simulink model "SC_Stage_Detail"  (R2026a)
settings: Solver=daessc  StopTime=Pd.Tend  MaxStep=1/(50*Pd.f)  RelTol=1e-5
undefined symbols (not defined in the file): Pd
libraries: fl_lib x8, nesl_utility x7, ee_lib x4
settings Model: Creator=highdreameater  LastModifiedBy=highdreameater

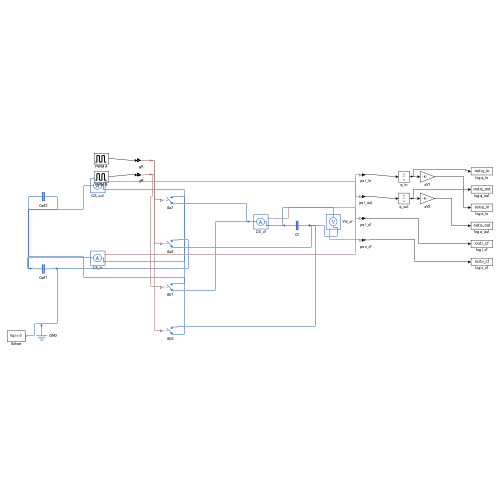
[thumbnail: Simulink's stored preview of the top-level diagram]
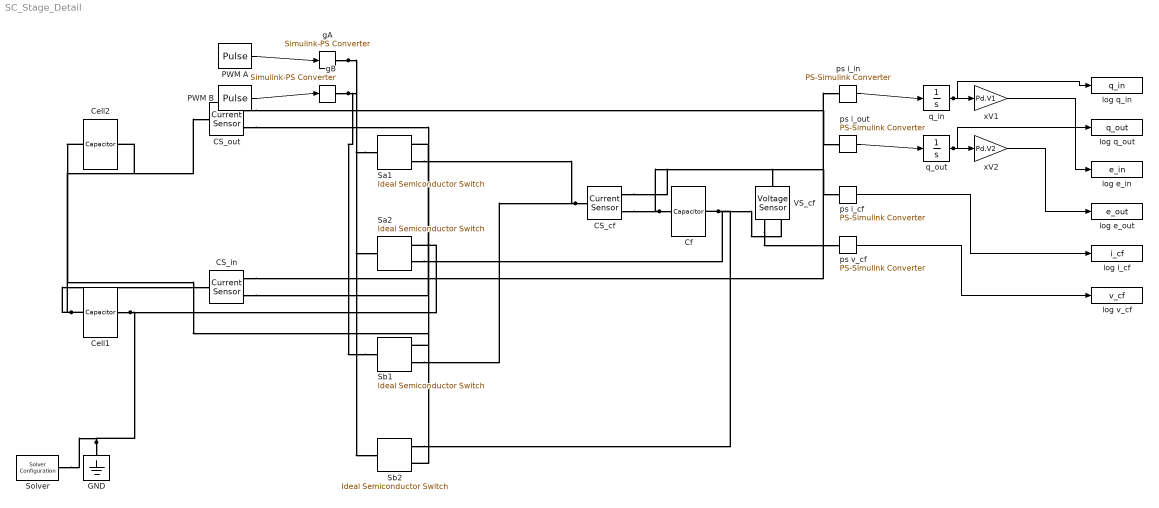
== system SC_Stage_Detail ==
  CS_cf : fl_lib/Electrical/Electrical Sensors/Current Sensor
  CS_in : fl_lib/Electrical/Electrical Sensors/Current Sensor
  CS_out : fl_lib/Electrical/Electrical Sensors/Current Sensor
  Cell1 : fl_lib/Electrical/Electrical Elements/Capacitor  c=Pd.C_emu F  r=Pd.ESR_emu Ohm  g=0 1/Ohm  i_specify=off  i_priority=None  i=0 A  i_nominal_specify=off  i_nominal_value=1  i_nominal_unit=A  v_specify=off  v_priority=None  v=0 V  v_nominal_specify=off  v_nominal_value=1  v_nominal_unit=V  vc_specify=on  vc_priority=High  vc=Pd.V1 V  vc_nominal_specify=off  vc_nominal_value=1  vc_nominal_unit=V
  Cell2 : fl_lib/Electrical/Electrical Elements/Capacitor  c=Pd.C_emu F  r=Pd.ESR_emu Ohm  g=0 1/Ohm  i_specify=off  i_priority=None  i=0 A  i_nominal_specify=off  i_nominal_value=1  i_nominal_unit=A  v_specify=off  v_priority=None  v=0 V  v_nominal_specify=off  v_nominal_value=1  v_nominal_unit=V  vc_specify=on  vc_priority=High  vc=Pd.V2 V  vc_nominal_specify=off  vc_nominal_value=1  vc_nominal_unit=V
  Cf : fl_lib/Electrical/Electrical Elements/Capacitor  c=Pd.C_fly F  r=Pd.ESR_fly Ohm  g=0 1/Ohm  i_specify=off  i_priority=None  i=0 A  i_nominal_specify=off  i_nominal_value=1  i_nominal_unit=A  v_specify=off  v_priority=None  v=0 V  v_nominal_specify=off  v_nominal_value=1  v_nominal_unit=V  vc_specify=on  vc_priority=High  vc=(Pd.V1+Pd.V2)/2 V  vc_nominal_specify=off  vc_nominal_value=1  vc_nominal_unit=V
  GND : fl_lib/Electrical/Electrical Elements/Electrical Reference
  PWM A : DiscretePulseGenerator  PulseType=Time based  Period=1/Pd.f  PulseWidth=Pd.duty_sc*100
  PWM B : DiscretePulseGenerator  PulseType=Time based  Period=1/Pd.f  PulseWidth=Pd.duty_sc*100  PhaseDelay=0.5/Pd.f
  Sa1 : ee_lib/Semiconductors & Converters/Ideal Semiconductor Switch  port_option=ee.enum.controlport.ps  Ron=Pd.R_on_sc Ohm  Goff=1e-9 1/Ohm  Vth=0.5 V  diode_param=ee.enum.semiconductors.protectionDiode.external  diode_Vf=0.8 V  diode_Ron=0.001 Ohm  diode_Goff=1e-5 1/Ohm  diode_C=50e-9 F  diode_iRM=-235 A  diode_iF=300 A  diode_idot=-50 A/us  diode_trr_param=ee.enum.converters.diodetrr.trr_factor  diode_trr_factor=3  diode_trr=15 us  diode_Qrr=1500 s*uA
  Sa2 : ee_lib/Semiconductors & Converters/Ideal Semiconductor Switch  port_option=ee.enum.controlport.ps  Ron=Pd.R_on_sc Ohm  Goff=1e-9 1/Ohm  Vth=0.5 V  diode_param=ee.enum.semiconductors.protectionDiode.external  diode_Vf=0.8 V  diode_Ron=0.001 Ohm  diode_Goff=1e-5 1/Ohm  diode_C=50e-9 F  diode_iRM=-235 A  diode_iF=300 A  diode_idot=-50 A/us  diode_trr_param=ee.enum.converters.diodetrr.trr_factor  diode_trr_factor=3  diode_trr=15 us  diode_Qrr=1500 s*uA
  Sb1 : ee_lib/Semiconductors & Converters/Ideal Semiconductor Switch  port_option=ee.enum.controlport.ps  Ron=Pd.R_on_sc Ohm  Goff=1e-9 1/Ohm  Vth=0.5 V  diode_param=ee.enum.semiconductors.protectionDiode.external  diode_Vf=0.8 V  diode_Ron=0.001 Ohm  diode_Goff=1e-5 1/Ohm  diode_C=50e-9 F  diode_iRM=-235 A  diode_iF=300 A  diode_idot=-50 A/us  diode_trr_param=ee.enum.converters.diodetrr.trr_factor  diode_trr_factor=3  diode_trr=15 us  diode_Qrr=1500 s*uA
  Sb2 : ee_lib/Semiconductors & Converters/Ideal Semiconductor Switch  port_option=ee.enum.controlport.ps  Ron=Pd.R_on_sc Ohm  Goff=1e-9 1/Ohm  Vth=0.5 V  diode_param=ee.enum.semiconductors.protectionDiode.external  diode_Vf=0.8 V  diode_Ron=0.001 Ohm  diode_Goff=1e-5 1/Ohm  diode_C=50e-9 F  diode_iRM=-235 A  diode_iF=300 A  diode_idot=-50 A/us  diode_trr_param=ee.enum.converters.diodetrr.trr_factor  diode_trr_factor=3  diode_trr=15 us  diode_Qrr=1500 s*uA
  Solver : nesl_utility/Solver Configuration  PhysicalDomain=network_engine_domain  SubClassName=solver  LeftPortType=input  RightPortType=generic  Tones=[]  Harmonics=[]  SimulateNoise=off  Profile=off  UseLocalSampling=off  EnableSwitchedLinearOptims=on  FrequencyDomain=off  UseCCode=off  RelTol=0.001  AbsTol=0.001  MinStep=1e-09  ToWorkspace=off  RevertToSquareIcSolve=off  NumHomotopyIterations=100  PhasorMode=off  PhasorModeNumHarmonics=1  ConsistencySolver=NEWTON_XTOL_AFTER_FTOL  CanonicalOrdering=CANONICAL  OptimizeIntermediates=OPTIMIZED  IndexReductionMethod=DerivativeReplacement  DoDC=off  ResidualTolerance=1e-09  ConsistencyTolSource=GLOBAL  ConsistencyAbsTol=0.001  ConsistencyRelTol=0.001  ConsistencyTolFactor=0.001  UseLocalSolver=off  LocalSolverChoice=NE_BACKWARD_EULER_ADVANCER  ResolveIndetEquations=on  FunctionEvalNumThread=1  LocalSolverSampleTime=0.001  DoFixedCost=off  MaxNonlinIter=3  MaxModeIter=2  ComputeImpulses=off  ImpulseIterations=2  LinearAlgebra=auto  LinearAlgebraNumThread=0  EquationFormulation=NE_TIME_EF  DelaysMemoryBudget=1024  AutomaticFiltering=on  FilteringTimeConstant=0.001  PartitionStorageMethod=AS_NEEDED  PartitionMemoryBudget=1024  PartitionMethod=ROBUST  MultibodyUseLocalSolver=off  MultibodyLocalSolverChoice=ODE1  MultibodyLocalSolverSampleTime=0.001
  VS_cf : fl_lib/Electrical/Electrical Sensors/Voltage Sensor
  gA : nesl_utility/Simulink-PS Converter  PhysicalDomain=network_engine_domain  SubClassName=ps_input  LeftPortType=input  RightPortType=output  PseudoPeriodic=off  Frequencies=[]  NoiseDistribution=none  NoiseParameters=[]  Unit=1  AffineConversion=off  FilteringAndDerivatives=provide  SimscapeFilterOrder=1  InputFilterTimeConstant=0.001  UdotUserProvided=0
  gB : nesl_utility/Simulink-PS Converter  PhysicalDomain=network_engine_domain  SubClassName=ps_input  LeftPortType=input  RightPortType=output  PseudoPeriodic=off  Frequencies=[]  NoiseDistribution=none  NoiseParameters=[]  Unit=1  AffineConversion=off  FilteringAndDerivatives=provide  SimscapeFilterOrder=1  InputFilterTimeConstant=0.001  UdotUserProvided=0
  log e_in : ToWorkspace  VariableName=e_in  SaveFormat=Timeseries  SampleTime=-1
  log e_out : ToWorkspace  VariableName=e_out  SaveFormat=Timeseries  SampleTime=-1
  log i_cf : ToWorkspace  VariableName=i_cf  SaveFormat=Timeseries  SampleTime=-1
  log q_in : ToWorkspace  VariableName=q_in  SaveFormat=Timeseries  SampleTime=-1
  log q_out : ToWorkspace  VariableName=q_out  SaveFormat=Timeseries  SampleTime=-1
  log v_cf : ToWorkspace  VariableName=v_cf  SaveFormat=Timeseries  SampleTime=-1
  ps i_cf : nesl_utility/PS-Simulink Converter  PhysicalDomain=network_engine_domain  SubClassName=ps_output  LeftPortType=input  RightPortType=output  PseudoPeriodic=off  Frequencies=[]  VectorFormat=inherit  Unit=A  AffineConversion=off
  ps i_in : nesl_utility/PS-Simulink Converter  PhysicalDomain=network_engine_domain  SubClassName=ps_output  LeftPortType=input  RightPortType=output  PseudoPeriodic=off  Frequencies=[]  VectorFormat=inherit  Unit=A  AffineConversion=off
  ps i_out : nesl_utility/PS-Simulink Converter  PhysicalDomain=network_engine_domain  SubClassName=ps_output  LeftPortType=input  RightPortType=output  PseudoPeriodic=off  Frequencies=[]  VectorFormat=inherit  Unit=A  AffineConversion=off
  ps v_cf : nesl_utility/PS-Simulink Converter  PhysicalDomain=network_engine_domain  SubClassName=ps_output  LeftPortType=input  RightPortType=output  PseudoPeriodic=off  Frequencies=[]  VectorFormat=inherit  Unit=V  AffineConversion=off
  q_in : Integrator
  q_out : Integrator
  xV1 : Gain  Gain=Pd.V1
  xV2 : Gain  Gain=Pd.V2
  wires:
  PWM A/1 -> gA/1
  PWM B/1 -> gB/1
  ps i_in/1 -> q_in/1
  ps i_out/1 -> q_out/1
  q_in/1 -> xV1/1, log q_in/1
  q_out/1 -> xV2/1, log q_out/1
  xV1/1 -> log e_in/1
  xV2/1 -> log e_out/1
  ps i_cf/1 -> log i_cf/1
  ps v_cf/1 -> log v_cf/1
  connections:
  GND/LConn1 -- Solver/RConn1 -- Cell1/RConn1 -- Sa2/RConn1
  Cell2/RConn1 -- Cell1/LConn1 -- CS_in/LConn1 -- CS_out/LConn1
  Sa1/LConn1 -- gA/RConn1 -- Sa2/LConn1
  Sb1/LConn1 -- gB/RConn1 -- Sb2/LConn1
  Cf/LConn1 -- CS_cf/RConn2 -- VS_cf/LConn1
  CS_in/RConn2 -- Sa1/RConn1
  CS_cf/LConn1 -- Sa1/RConn2 -- Sb1/RConn2
  Sa2/RConn2 -- Sb2/RConn1 -- Cf/RConn1 -- VS_cf/RConn2
  Cell2/LConn1 -- Sb1/RConn1
  CS_out/RConn2 -- Sb2/RConn2
  CS_in/RConn1 -- ps i_in/LConn1
  CS_out/RConn1 -- ps i_out/LConn1
  CS_cf/RConn1 -- ps i_cf/LConn1
  VS_cf/RConn1 -- ps v_cf/LConn1
